simulink model "emulater"  (R2024b)
settings: Solver=FixedStepDiscrete  StartTime=0.0  StopTime=inf  FixedStep=0.01  RelTol=1e-3  EnableMultiTasking=on
libraries: arduinolib x12
settings Model: ExtModeTrigDuration=2  Creator=39389  LastModifiedBy=39389
settings SolverCC: AutoInsertRateTranBlk=on
settings OptimizationCC: EnhancedBackFolding=on  PassReuseOutputArgsAs=Individual arguments  ZeroExternalMemoryAtStartup=off  ZeroInternalMemoryAtStartup=off  MaxStackSize=64  OptimizeBlockOrder=speed  DifferentSizesBufferReuse=on  OptimizationCustomize=off  EfficientTunableParamExpr=on
settings DebuggingCC: ParameterTunabilityLossMsg=error
settings HardwareCC: ProdBitPerInt=16  ProdBitPerPointer=16  ProdBitPerSizeT=16  ProdBitPerPtrDiffT=16  ProdLargestAtomicFloat=None  ProdWordSize=8  ProdHWDeviceType=Atmel->AVR
settings SFSimCC: MATLABDynamicMemAlloc=off
settings RTWCC: Description=Embedded Coder  SystemTargetFile=ert.tlc  HardwareBoard=Arduino Uno  TemplateMakefile=ert_default_tmf  Toolchain=Arduino AVR  BuildConfiguration=Faster Runs
settings CodeAppCC: ForceParamTrailComments=on  IgnoreCustomStorageClasses=off  OperatorAnnotations=on  SimulinkDataObjDesc=on  SFDataObjDesc=on  InsertBlockDesc=on
settings ERTTargetCC: TargetLangStandard=C99 (ISO)  SupportContinuousTime=on  SupportVariableSizeSignals=on  ExtModeTransport=3  ExtModeStaticAlloc=on  ExtModeAutomaticAllocSize=off  ExtModeStaticAllocSize=250  ExtModeMexFile=ext_xcp  ExtModeIntrfLevel=Level2 - Open  InlinedParameterPlacement=Hierarchical

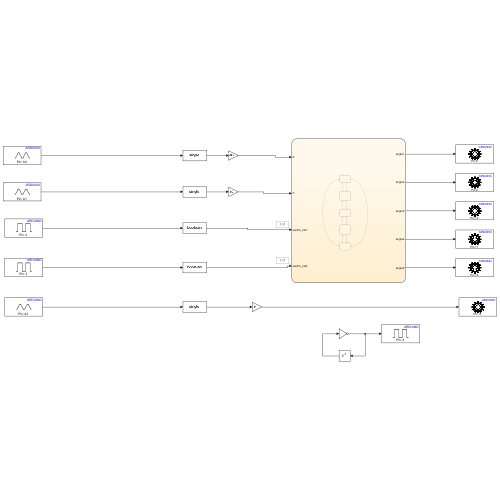
[thumbnail: Simulink's stored preview of the top-level diagram]
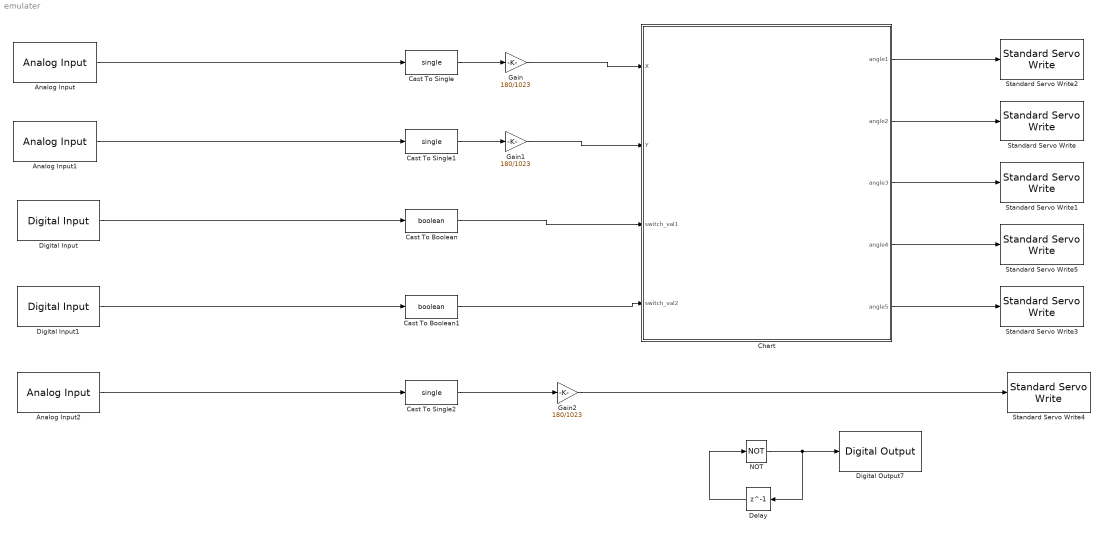
== system emulater ==
  Analog Input : arduinolib/Analog Input  pinNumber=0  ReadResultsOnly=off  ConversionTriggerSource=Software  ExternalTriggerType=uint32( 0 )  OutputDataType=uint16  EnableConversionCompleteNotify=off  EnableOuputStatus=off  SampleTime=-1  blockPlatform=arduino
      settings: SourceProductName=Common
  Analog Input1 : arduinolib/Analog Input  pinNumber=1  ReadResultsOnly=off  ConversionTriggerSource=Software  ExternalTriggerType=uint32( 0 )  OutputDataType=uint16  EnableConversionCompleteNotify=off  EnableOuputStatus=off  SampleTime=-1  blockPlatform=arduino
      settings: SourceProductName=Common
  Analog Input2 : arduinolib/Analog Input  pinNumber=3  ReadResultsOnly=off  ConversionTriggerSource=Software  ExternalTriggerType=uint32( 0 )  OutputDataType=uint16  EnableConversionCompleteNotify=off  EnableOuputStatus=off  SampleTime=-1  blockPlatform=arduino
      settings: SourceProductName=Common
  Cast To Boolean : DataTypeConversion  OutDataTypeStr=boolean  SaturateOnIntegerOverflow=off  RndMeth=Floor
  Cast To Boolean1 : DataTypeConversion  OutDataTypeStr=boolean  SaturateOnIntegerOverflow=off  RndMeth=Floor
  Cast To Single : DataTypeConversion  OutDataTypeStr=single  SaturateOnIntegerOverflow=off  RndMeth=Floor
  Cast To Single1 : DataTypeConversion  OutDataTypeStr=single  SaturateOnIntegerOverflow=off  RndMeth=Floor
  Cast To Single2 : DataTypeConversion  OutDataTypeStr=single  SaturateOnIntegerOverflow=off  RndMeth=Floor
  Chart : Stateflow chart  TreatAsAtomicUnit=on
  Delay : Delay  DelayLength=1  SampleTime=0.01
  Digital Input : arduinolib/Digital Input  pinNumber=2  mode=Default  Direction=input  SampleTime=0.1  blockPlatform=arduino
      settings: SourceProductName=Common
  Digital Input1 : arduinolib/Digital Input  pinNumber=3  mode=Default  Direction=input  SampleTime=0.1  blockPlatform=arduino
      settings: SourceProductName=Common
  Digital Output7 : arduinolib/Digital Output  pinNumber=4  Direction=output  blockPlatform=arduino
      settings: SourceProductName=Common
  Gain : Gain  Gain=180/1023
  Gain1 : Gain  Gain=180/1023
  Gain2 : Gain  Gain=180/1023
  NOT : Logic  Operator=NOT  IconShape=distinctive  AllPortsSameDT=off  OutDataTypeStr=boolean
  Standard Servo Write : arduinolib/Standard Servo Write  pinNumber=9  ServoIndex=0  blockPlatform=ARDUINO
      settings: SourceProductName=Common
  Standard Servo Write1 : arduinolib/Standard Servo Write  pinNumber=10  ServoIndex=1  blockPlatform=ARDUINO
      settings: SourceProductName=Common
  Standard Servo Write2 : arduinolib/Standard Servo Write  pinNumber=8  ServoIndex=2  blockPlatform=ARDUINO
      settings: SourceProductName=Common
  Standard Servo Write3 : arduinolib/Standard Servo Write  pinNumber=12  ServoIndex=3  blockPlatform=ARDUINO
      settings: SourceProductName=Common
  Standard Servo Write4 : arduinolib/Standard Servo Write  pinNumber=13  ServoIndex=4  blockPlatform=ARDUINO
      settings: SourceProductName=Common
  Standard Servo Write5 : arduinolib/Standard Servo Write  pinNumber=11  ServoIndex=5  blockPlatform=ARDUINO
      settings: SourceProductName=Common
  wires:
  Analog Input2/1 -> Cast To Single2/1
  Cast To Single2/1 -> Gain2/1
  Digital Input1/1 -> Cast To Boolean1/1
  Analog Input1/1 -> Cast To Single1/1
  Analog Input/1 -> Cast To Single/1
  Cast To Boolean1/1 -> Chart/4(switch_val2)
  Cast To Single1/1 -> Gain1/1
  Gain1/1 -> Chart/2(Y)
  Digital Input/1 -> Cast To Boolean/1
  Cast To Single/1 -> Gain/1
  Gain/1 -> Chart/1(X)
  Chart/1(angle1) -> Standard Servo Write2/1
  Chart/2(angle2) -> Standard Servo Write/1
  Chart/3(angle3) -> Standard Servo Write1/1
  Chart/4(angle4) -> Standard Servo Write5/1
  Chart/5(angle5) -> Standard Servo Write3/1
  Gain2/1 -> Standard Servo Write4/1
  Cast To Boolean/1 -> Chart/3(switch_val1)
  Delay/1 -> NOT/1
  NOT/1 -> Delay/1, Digital Output7/1

== stateflow chart emulater/Chart ==
  settings: updateMethod=DISCRETE  sampleTime=0.01
  state servo1
    during:
    angle1=X;
  state servo2
    during:
    angle2=Y;
  state servo3
    during:
    angle3=Y;
  state servo4
    during:
    angle4=X;
  state servo5
    during:
    angle5=Y;
  (default) -> servo1
  servo1 -> servo5 [order 2] : [switch_val2 == 1 && after(1, sec)]
  servo5 -> servo1 [order 1] : [switch_val1 == 1 && after(1, sec)]
  servo2 -> servo1 [order 2] : [switch_val2 == 1 && after(1, sec)]
  servo1 -> servo2 [order 1] : [switch_val1 == 1 && after(1, sec)]
  servo3 -> servo2 [order 2] : [switch_val2 == 1 && after(1, sec)]
  servo2 -> servo3 [order 1] : [switch_val1 == 1 && after(1, sec)]
  servo4 -> servo3 [order 2] : [switch_val2 == 1 && after(1, sec)]
  servo3 -> servo4 [order 1] : [switch_val1 == 1 && after(1, sec)]
  servo5 -> servo4 [order 2] : [switch_val2 == 1 && after(1, sec)]
  servo4 -> servo5 [order 1] : [switch_val1 == 1 && after(1, sec)]
  data: X input; Y input; switch_val1 input; angle1 output; angle2 output; angle3 output; angle4 output; angle5 output; switch_val2 input
